simulink model "can2_mcu_status_pack"  (R2026b)
settings: Solver=VariableStepAuto
undefined symbols (not defined in the file or in its folder): P
libraries: simulink x1, svdutilitieslib x1
settings Model: Creator=aomar  LastModifiedBy=aomar

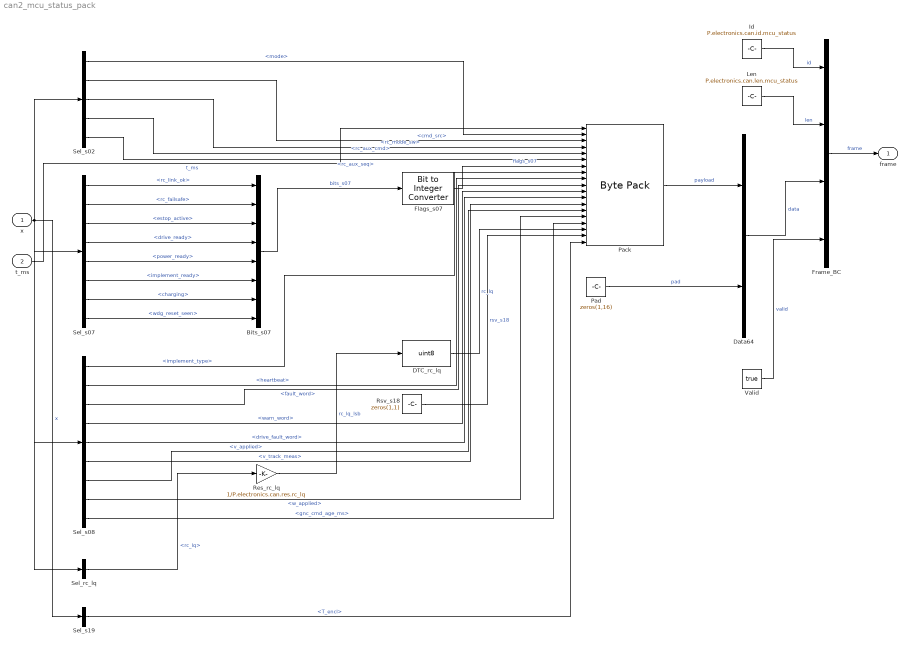
== system can2_mcu_status_pack ==
  x : Inport  OutDataTypeStr=Bus: Bus_McuStatus
  t_ms : Inport  Port=2  OutDataTypeStr=uint32
  Bits_s07 : Concatenate  NumInputs=8
  DTC_rc_lq : DataTypeConversion  OutDataTypeStr=uint8  RndMeth=Round
  Data64 : Concatenate
  Flags_s07 : simulink/Logic and Bit Operations/Bit to Integer Converter  nbits=8  bitOrder=LSB first  signedOutputValues=Unsigned  outDtype=uint8  outDtypeSigned=Inherit via internal rule
      settings: LibrarySourceBlock=|
      | commutil2/Bit to Integer
      | Converter
  Frame_BC : BusCreator  Inputs=4  OutDataTypeStr=Bus: Bus_CanFrame64  NonVirtualBus=on
      settings: InheritFromInputs=off
  Id : Constant  Value=P.electronics.can.id.mcu_status  OutDataTypeStr=uint32  SampleTime=-1
  Len : Constant  Value=P.electronics.can.len.mcu_status  OutDataTypeStr=uint8  SampleTime=-1
  Pack : svdutilitieslib/Byte Pack  maskPackedDataType=uint8  datatypes={'uint32','uint8','uint8','uint8','uint8','uint8','uint8','uint8','uint8','uint32','uint32','uint32','single','single','single','uint16','uint8','uint8','single'}  byteAlign=1  blockPlatform=arduinoert
      settings: LibrarySourceBlock=mcblib/Signal Management/Byte Pack
  Pad : Constant  Value=zeros(1,16)  OutDataTypeStr=uint8  SampleTime=-1
  Res_rc_lq : Gain  Gain=1/P.electronics.can.res.rc_lq
  Rsv_s18 : Constant  Value=zeros(1,1)  OutDataTypeStr=uint8  SampleTime=-1
  Sel_rc_lq : BusSelector  OutputSignals=rc_lq
  Sel_s02 : BusSelector  OutputSignals=mode,cmd_src,rc_mode_sw,rc_aux_cmd,rc_aux_seq
  Sel_s07 : BusSelector  OutputSignals=rc_link_ok,rc_failsafe,estop_active,drive_ready,power_ready,implement_ready,charging,wdg_reset_seen
  Sel_s08 : BusSelector  OutputSignals=implement_type,heartbeat,fault_word,warn_word,drive_fault_word,v_track_meas,v_applied,w_applied,gnc_cmd_age_ms
  Sel_s19 : BusSelector  OutputSignals=T_encl
  Valid : Constant  Value=true  OutDataTypeStr=boolean  SampleTime=-1
  frame : Outport  OutDataTypeStr=Bus: Bus_CanFrame64
  wires:
  x/1 -> Sel_s19/1, Sel_rc_lq/1, Sel_s08/1, Sel_s02/1, Sel_s07/1  "x"
  t_ms/1 -> Pack/1  "t_ms"
  Sel_s02/1 -> Pack/2  "<mode>"
  Sel_s02/2 -> Pack/3  "<cmd_src>"
  Sel_s02/3 -> Pack/4  "<rc_mode_sw>"
  Sel_s02/4 -> Pack/5  "<rc_aux_cmd>"
  Sel_s02/5 -> Pack/6  "<rc_aux_seq>"
  Sel_s07/1 -> Bits_s07/1  "<rc_link_ok>"
  Sel_s07/2 -> Bits_s07/2  "<rc_failsafe>"
  Sel_s07/3 -> Bits_s07/3  "<estop_active>"
  Sel_s07/4 -> Bits_s07/4  "<drive_ready>"
  Sel_s07/5 -> Bits_s07/5  "<power_ready>"
  Sel_s07/6 -> Bits_s07/6  "<implement_ready>"
  Sel_s07/7 -> Bits_s07/7  "<charging>"
  Sel_s07/8 -> Bits_s07/8  "<wdg_reset_seen>"
  Sel_s08/1 -> Pack/8  "<implement_type>"
  Sel_s08/2 -> Pack/9  "<heartbeat>"
  Sel_s08/3 -> Pack/10  "<fault_word>"
  Sel_s08/4 -> Pack/11  "<warn_word>"
  Sel_s08/5 -> Pack/12  "<drive_fault_word>"
  Sel_s08/6 -> Pack/13  "<v_track_meas>"
  Sel_s08/7 -> Pack/14  "<v_applied>"
  Sel_s08/8 -> Pack/15  "<w_applied>"
  Sel_s08/9 -> Pack/16  "<gnc_cmd_age_ms>"
  Sel_rc_lq/1 -> Res_rc_lq/1  "<rc_lq>"
  Sel_s19/1 -> Pack/19  "<T_encl>"
  Bits_s07/1 -> Flags_s07/1  "bits_s07"
  Res_rc_lq/1 -> DTC_rc_lq/1  "rc_lq_lsb"
  Rsv_s18/1 -> Pack/18  "rsv_s18"
  DTC_rc_lq/1 -> Pack/17  "rc_lq"
  Flags_s07/1 -> Pack/7  "flags_s07"
  Pad/1 -> Data64/2  "pad"
  Pack/1 -> Data64/1  "payload"
  Data64/1 -> Frame_BC/3  "data"
  Id/1 -> Frame_BC/1  "id"
  Len/1 -> Frame_BC/2  "len"
  Valid/1 -> Frame_BC/4  "valid"
  Frame_BC/1 -> frame/1  "frame"
